simulink model "arducopter"  (R2024b)
settings: Solver=FixedStepAuto  StartTime=0.0  StopTime=simIn.param.timeEnd  FixedStep=simIn.param.dt  RelTol=1e-3
undefined symbols (not defined in the file or in its folder): DiscIntNeverNeededParam, sim, simIn
libraries: simulink x60, slident x4, vrlib x1
(part 5 of 9)

== system arducopter/Position Controller/PID Velocity z/I ==
  note: Integrator, see AC_PID_Basic::update_i()
      | Initialization: integrator=0 (see AC_PosControl::init_z())
  e : Inport
  limitNeg : Inport  Port=2
  limitPos : Inport  Port=3
  ki : Inport  Port=4
  i_max : Inport  Port=5
  Constant1 : Constant  Value=simIn.param.dt
  Data Type Conversion1 : DataTypeConversion  OutDataTypeStr=single  SaturateOnIntegerOverflow=off  RndMeth=Floor
  IC1 : InitialCondition  Value=0
  Integrator : MATLAB Function  TreatAsAtomicUnit=on
  Unit Delay1 : UnitDelay  InitialCondition=single(0)  SampleTime=-1  HasFrameUpgradeWarning=on
  integrator : Outport
  wires:
  e/1 -> Integrator/1(error)
  Integrator/1(integrator_out) -> IC1/1
  [integrator_out] -> integrator/1
  Constant1/1 -> Data Type Conversion1/1
  limitNeg/1 -> Integrator/3(limitNeg)
  [integrator_out] -> Unit Delay1/1
  IC1/1 -> [integrator_out]
  Unit Delay1/1 -> Integrator/2(integrator)
  ki/1 -> Integrator/5(ki)
  i_max/1 -> Integrator/6(i_max)
  Data Type Conversion1/1 -> Integrator/7(dt)
  limitPos/1 -> Integrator/4(limitPos)

== system arducopter/Position Controller/PID Velocity z/RAT_FLTD ==
  note: Digital Filter:
      | $y_n = (1 - \alpha)y_{n-1} + x \cdot \alpha$
  note: Alpha Calculation:
      | $\alpha = \frac{\mathrm{d}t}{\mathrm{d}t + 2 \pi f_{\mathrm{Cutoff}}$
  note: See AC_PID_Basics.cpp, update_all()
  note: See AP_Math.cpp, calc_lowpass_alpha_dt()
  u : Inport
  cutoff_freq : Inport  Port=2
  ATC input time constant : Constant  Value=simIn.param.dt
  Add : Sum
  Calculate Alpha : Product  Inputs=*/
  Compare To Zero : simulink/Logic and Bit Operations/Compare To Zero  relop=<=  OutDataTypeStr=boolean
  Compare To Zero1 : simulink/Logic and Bit Operations/Compare To Zero  relop=<=  OutDataTypeStr=boolean
  Constant2 : Constant  OutDataTypeStr=single
  Constant3 : Constant  OutDataTypeStr=single
  Constant4 : Constant  OutDataTypeStr=single
  Data Type Conversion1 : DataTypeConversion  OutDataTypeStr=single  SaturateOnIntegerOverflow=off  RndMeth=Floor
  Divide : Product  Inputs=*/
  Gain : Gain  Gain=2*pi
  IC : InitialCondition  Value=0
  Logical Operator : Logic  Operator=OR  AllPortsSameDT=off  OutDataTypeStr=boolean
  Product : Product
  Product1 : Product
  Subtract1 : Sum  Inputs=+-
  Sum : Sum  Inputs=++|  OutDataTypeStr=single
  Switch : Switch  Criteria=u2 > Threshold  SaturateOnIntegerOverflow=off  InputSameDT=off
  Unit Delay : UnitDelay  SampleTime=-1  HasFrameUpgradeWarning=on
  y : Outport
  wires:
  Product1/1 -> Sum/2
  Unit Delay/1 -> Product1/2
  Subtract1/1 -> Product1/1
  [alpha] -> Subtract1/2
  Constant2/1 -> Subtract1/1
  [alpha] -> Product/1
  Calculate Alpha/1 -> Switch/3
  Add/1 -> Calculate Alpha/2
  [dt] -> Add/1, Calculate Alpha/1
  Gain/1 -> Divide/2
  cutoff_freq/1 -> [cutoff_freq]
  u/1 -> Product/2
  Divide/1 -> Add/2
  Constant3/1 -> Divide/1
  Product/1 -> Sum/1
  Switch/1 -> [alpha]
  ATC input time constant/1 -> Data Type Conversion1/1
  [cutoff_freq] -> Gain/1
  [dt] -> Compare To Zero/1
  [cutoff_freq] -> Compare To Zero1/1
  Compare To Zero/1 -> Logical Operator/1
  Compare To Zero1/1 -> Logical Operator/2
  Logical Operator/1 -> Switch/2
  Constant4/1 -> Switch/1
  Sum/1 -> IC/1
  IC/1 -> Unit Delay/1, y/1
  Data Type Conversion1/1 -> [dt]

== system arducopter/Position Controller/PID Velocity z/RAT_FLTE ==
  note: Digital Filter:
      | $y_n = (1 - \alpha)y_{n-1} + x \cdot \alpha$
  note: Alpha Calculation:
      | $\alpha = \frac{\mathrm{d}t}{\mathrm{d}t + 2 \pi f_{\mathrm{Cutoff}}$
  note: See AC_PID_Basic.cpp, update_all()
  note: See AP_Math.cpp, calc_lowpass_alpha_dt()
  u : Inport
  cutoff_freq : Inport  Port=2
  ATC input time constant : Constant  Value=simIn.param.dt
  Add : Sum
  Calculate Alpha : Product  Inputs=*/
  Compare To Zero : simulink/Logic and Bit Operations/Compare To Zero  relop=<=  OutDataTypeStr=boolean
  Compare To Zero1 : simulink/Logic and Bit Operations/Compare To Zero  relop=<=  OutDataTypeStr=boolean
  Constant2 : Constant  OutDataTypeStr=single
  Constant3 : Constant  OutDataTypeStr=single
  Constant4 : Constant  OutDataTypeStr=single
  Data Type Conversion1 : DataTypeConversion  OutDataTypeStr=single  SaturateOnIntegerOverflow=off  RndMeth=Floor
  Divide : Product  Inputs=*/
  Gain : Gain  Gain=2*pi
  IC : InitialCondition  Value=0
  Logical Operator : Logic  Operator=OR  AllPortsSameDT=off  OutDataTypeStr=boolean
  Product : Product
  Product1 : Product
  Subtract1 : Sum  Inputs=+-
  Sum : Sum  Inputs=++|  OutDataTypeStr=single
  Switch : Switch  Criteria=u2 > Threshold  SaturateOnIntegerOverflow=off  InputSameDT=off
  Unit Delay : UnitDelay  SampleTime=-1  HasFrameUpgradeWarning=on
  y : Outport
  wires:
  Product1/1 -> Sum/2
  Unit Delay/1 -> Product1/2
  Subtract1/1 -> Product1/1
  [alpha] -> Subtract1/2
  Constant2/1 -> Subtract1/1
  [alpha] -> Product/1
  Calculate Alpha/1 -> Switch/3
  Add/1 -> Calculate Alpha/2
  [dt] -> Add/1, Calculate Alpha/1
  Gain/1 -> Divide/2
  cutoff_freq/1 -> [cutoff_freq]
  u/1 -> Product/2
  Divide/1 -> Add/2
  Constant3/1 -> Divide/1
  Product/1 -> Sum/1
  Switch/1 -> [alpha]
  ATC input time constant/1 -> Data Type Conversion1/1
  [cutoff_freq] -> Gain/1
  [dt] -> Compare To Zero/1
  [cutoff_freq] -> Compare To Zero1/1
  Compare To Zero/1 -> Logical Operator/1
  Compare To Zero1/1 -> Logical Operator/2
  Logical Operator/1 -> Switch/2
  Constant4/1 -> Switch/1
  Sum/1 -> IC/1
  IC/1 -> Unit Delay/1, y/1
  Data Type Conversion1/1 -> [dt]

== system arducopter/Position Controller/PID Velocity z/Scale Factor Z ==
  note: AP_AHRS::getControlScaleZ()
      | This subsystem calculates a scaling factor for the target of vertical motion quantities based on the EKF type that is being used.
      | Taken from AP_AHRS::getControlScaleZ() in AP_AHRS.cpp. Called in AC_PosControl::update_z_controller().
      | Flying with only DCM lower the gain of the controllers by 4x to cope with high lag.
  ekfType : Inport
  EKF used : Constant  OutDataTypeStr=single
  No EKF : Constant  Value=0.25  OutDataTypeStr=single
  Switch : Switch  Criteria=u2 > Threshold  SaturateOnIntegerOverflow=off  InputSameDT=off
  scale_z : Outport
  wires:
  ekfType/1 -> Switch/2
  EKF used/1 -> Switch/1
  No EKF/1 -> Switch/3
  Switch/1 -> scale_z/1

== system arducopter/Position Controller/calc des climb rate/constrain climb rate ==
  note: Based on get_pilot_speed_dn()
      | Use maximum up-speed if down-speed limit is 0
  in : Inport
  Abs : Abs  SaturateOnIntegerOverflow=off
  Abs1 : Abs  SaturateOnIntegerOverflow=off
  Constant1 : Constant  Value=simIn.param.PSCD.VEL_MAX_DN
  Constant2 : Constant  Value=simIn.param.PSCD.VEL_MAX_UP
  Constant3 : Constant  Value=simIn.param.PSCD.VEL_MAX_UP
  Gain : Gain  Gain=-1
  Saturation Dynamic : simulink/Discontinuities/Saturation Dynamic  OutMin=[]  OutMax=[]  OutDataTypeStr=Inherit: Same as second input  OutDataType=fixdt(1, 16)  OutScaling=2^-10  DoSatur=off
  Switch : Switch  Criteria=u2 > Threshold  SaturateOnIntegerOverflow=off  InputSameDT=off
  out : Outport
  wires:
  Constant1/1 -> Abs/1, Switch/2
  Constant2/1 -> Abs1/1
  Abs/1 -> Switch/1
  Abs1/1 -> Switch/3
  Saturation Dynamic/1 -> out/1
  Switch/1 -> Gain/1
  Gain/1 -> Saturation Dynamic/3
  in/1 -> Saturation Dynamic/2
  Constant3/1 -> Saturation Dynamic/1

== system arducopter/Position Controller/set_pos_target_z_from_climb_rate()/input_vel_accel_z ==
  note: input_vel_accel_z()
      | This subsystem takes the current target position (posTarIn) and desired velocity and acceleration (velDesTar and accDesTar).
      | First, it updates the target position and desired velocity based on the current desired acceleration (accDesIn) (1).
      | Secondly, it calculates the required jerk limited adjustment to the acceleration for the next time dt (accDes) to reach the desired velocity and acceleration targets (velDesTar and accDesTar) (2).
  note: (2) shape_vel_accel()
      | Adjustment of the desired acceleration to follow a jerk limited kinematic path to vel and acc
  note: (1) update_pos_vel_accel()
      | Adjust desired position and velocity based on desired acceleration
  note: Calculate overspeed gain to calculate increased max accel and jerk if over speed
  velDesTar : Inport
  accDesTar : Inport  Port=2
  limitVectorZ : Inport  Port=3
  velMaxUp : Inport  Port=4
  velMaxDn : Inport  Port=5
  accMaxZ : Inport  Port=6
  jerkMax : Inport  Port=7
  posTarIn : Inport  Port=8
  posErr : Inport  Port=9
  velErr : Inport  Port=10
  velDesIn : Inport  Port=11
  accDesIn : Inport  Port=12
  Constant : Constant  Value=simIn.param.PSCD.OVERSPEED_GAIN_Z
  Constant1 : Constant  OutDataTypeStr=boolean
  Constant2 : Constant  Value=simIn.param.dt  OutDataTypeStr=single
  MATLAB Function : MATLAB Function  TreatAsAtomicUnit=on
  Product : Product
  Product1 : Product
  calc accMin : Subsystem
  shape_vel_accel : Subsystem
  update_pos_vel_accel : Subsystem
  posTar : Outport
  velDes : Outport  Port=2
  accDes : Outport  Port=3
  wires:
  velMaxUp/1 -> MATLAB Function/1(velMaxUp)
  accMaxZ/1 -> Product/2
  velDesIn/1 -> [velDesIn]
  velMaxDn/1 -> MATLAB Function/2(velMaxDn)
  Constant/1 -> MATLAB Function/4(overspeedGainDefault)
  [velDesIn] -> MATLAB Function/3(velDes)
  posTarIn/1 -> update_pos_vel_accel/1(posTarIn)
  [velDesIn] -> update_pos_vel_accel/2(velDesIn)
  accDesIn/1 -> [accDesIn]
  limitVectorZ/1 -> update_pos_vel_accel/4(limitVectorZ)
  update_pos_vel_accel/2(velDes) -> [velDes]
  accDesTar/1 -> shape_vel_accel/2(acc)
  velDesTar/1 -> shape_vel_accel/1(vel)
  [accDesIn] -> update_pos_vel_accel/3(accDesIn)
  [accDesIn] -> shape_vel_accel/4(accDes)
  [accMax] -> calc accMin/1(accMax), shape_vel_accel/6(accMax)
  calc accMin/1(accMin) -> shape_vel_accel/5(accMin)
  Constant2/1 -> shape_vel_accel/8(dt)
  Constant1/1 -> shape_vel_accel/9(limitTotalAccel)
  update_pos_vel_accel/1(posTar) -> posTar/1
  [velDes] -> shape_vel_accel/3(velDes)
  [velDes] -> velDes/1
  shape_vel_accel/1(accDesShaped) -> accDes/1
  MATLAB Function/1(overspeedGain) -> Product1/1, Product/1
  Product/1 -> [accMax]
  jerkMax/1 -> Product1/2
  Product1/1 -> [jerkMax]
  [jerkMax] -> shape_vel_accel/7(jerkMax)
  posErr/1 -> update_pos_vel_accel/5(posErr)
  velErr/1 -> update_pos_vel_accel/6(velErr)

== system arducopter/Rate Controller/PID Pitch Rate/Calc Derivative ==
  e : Inport
  ATC input time constant : Constant  Value=simIn.param.dt
  Data Type Conversion : DataTypeConversion  OutDataTypeStr=single  SaturateOnIntegerOverflow=off  RndMeth=Floor
  Divide : Product  Inputs=*/
  Sum : Sum  Inputs=|+-
  Unit Delay : UnitDelay  SampleTime=-1  HasFrameUpgradeWarning=on
  derivative : Outport
  wires:
  e/1 -> Sum/1, Unit Delay/1
  Unit Delay/1 -> Sum/2
  Sum/1 -> Divide/1
  ATC input time constant/1 -> Data Type Conversion/1
  Divide/1 -> derivative/1
  Data Type Conversion/1 -> Divide/2

== system arducopter/Rate Controller/PID Pitch Rate/I ==
  note: Integrator, see AC_PID::update_i()
  e : Inport
  limit_flg : Inport  Port=2
  ki : Inport  Port=3
  i_max : Inport  Port=4
  Constant1 : Constant  Value=simIn.param.dt
  Data Type Conversion : DataTypeConversion  OutDataTypeStr=single  SaturateOnIntegerOverflow=off  RndMeth=Floor
  IC1 : InitialCondition  Value=simIn.init.PIDP.I
  Integrator : MATLAB Function  TreatAsAtomicUnit=on
  Unit Delay1 : UnitDelay  SampleTime=-1  HasFrameUpgradeWarning=on
  integrator : Outport
  wires:
  [integrator_out] -> integrator/1
  Constant1/1 -> Data Type Conversion/1
  limit_flg/1 -> Integrator/3(limit_flg)
  [integrator_out] -> Unit Delay1/1
  IC1/1 -> [integrator_out]
  Unit Delay1/1 -> Integrator/2(integrator)
  ki/1 -> Integrator/4(ki)
  i_max/1 -> Integrator/5(i_max)
  e/1 -> Integrator/1(error)
  Integrator/1(integrator_out) -> IC1/1
  Data Type Conversion/1 -> Integrator/6(dt)

== system arducopter/Rate Controller/PID Pitch Rate/RAT_FLTD ==
  note: Digital Filter:
      | $y_n = (1 - \alpha)y_{n-1} + x \cdot \alpha$
  note: See AC_PID.cpp, update_all()
  note: See AP_Math.cpp, calc_lowpass_alpha_dt()
  note: Alpha Calculation:
      | $\alpha = \frac{\mathrm{d}t}{\mathrm{d}t + 2 \pi f_{\mathrm{Cutoff}}$
  u : Inport
  cutoff_freq : Inport  Port=2
  ATC input time constant1 : Constant  Value=simIn.param.dt
  Add1 : Sum
  Calculate Alpha1 : Product  Inputs=*/
  Compare To Zero2 : simulink/Logic and Bit Operations/Compare To Zero  relop=<=  OutDataTypeStr=boolean
  Compare To Zero3 : simulink/Logic and Bit Operations/Compare To Zero  relop=<=  OutDataTypeStr=boolean
  Compare To Zero4 : simulink/Logic and Bit Operations/Compare To Zero  relop=~=  OutDataTypeStr=boolean
  Constant1 : Constant  OutDataTypeStr=single
  Constant2 : Constant  OutDataTypeStr=single
  Constant5 : Constant  OutDataTypeStr=single
  Data Type Conversion1 : DataTypeConversion  OutDataTypeStr=single  SaturateOnIntegerOverflow=off  RndMeth=Floor
  Divide1 : Product  Inputs=*/
  Gain1 : Gain  Gain=2*pi
  IC : InitialCondition  Value=simIn.init.PIDP.DerFilt
  Logical Operator1 : Logic  Operator=OR  AllPortsSameDT=off  OutDataTypeStr=boolean
  Product : Product
  Product1 : Product
  Product2 : Product
  Subtract1 : Sum  Inputs=+-
  Sum : Sum  Inputs=++|  AccumDataTypeStr=single
  Switch1 : Switch  Criteria=u2 > Threshold  SaturateOnIntegerOverflow=off  InputSameDT=off
  Unit Delay : UnitDelay  SampleTime=-1  HasFrameUpgradeWarning=on
  y : Outport
  wires:
  Product1/1 -> Sum/2
  Unit Delay/1 -> Product1/2
  Subtract1/1 -> Product1/1
  [alpha] -> Subtract1/2
  Constant2/1 -> Subtract1/1
  [alpha] -> Product/1
  u/1 -> Product/2
  Product/1 -> Sum/1
  Sum/1 -> IC/1
  IC/1 -> Unit Delay/1, y/1
  [dt] -> Compare To Zero2/1
  Constant1/1 -> Divide1/1
  Divide1/1 -> Add1/2
  Product2/1 -> Switch1/1
  Add1/1 -> Calculate Alpha1/2
  Gain1/1 -> Divide1/2
  Compare To Zero3/1 -> Logical Operator1/2
  [dt] -> Compare To Zero4/1
  Data Type Conversion1/1 -> [dt]
  ATC input time constant1/1 -> Data Type Conversion1/1
  [cutoff_freq] -> Gain1/1
  Switch1/1 -> [alpha]
  [dt] -> Calculate Alpha1/1, Add1/1
  Compare To Zero4/1 -> Product2/1
  cutoff_freq/1 -> [cutoff_freq]
  Compare To Zero2/1 -> Logical Operator1/1
  [cutoff_freq] -> Compare To Zero3/1
  Calculate Alpha1/1 -> Switch1/3
  Logical Operator1/1 -> Switch1/2
  Constant5/1 -> Product2/2

== system arducopter/Rate Controller/PID Pitch Rate/RAT_FLTE ==
  note: Digital Filter:
      | $y_n = (1 - \alpha)y_{n-1} + x \cdot \alpha$
  note: See AC_PID.cpp, update_all()
  note: See AP_Math.cpp, calc_lowpass_alpha_dt()
  note: Alpha Calculation:
      | $\alpha = \frac{\mathrm{d}t}{\mathrm{d}t + 2 \pi f_{\mathrm{Cutoff}}$
  u : Inport
  cutoff_freq : Inport  Port=2
  ATC input time constant1 : Constant  Value=simIn.param.dt
  Add1 : Sum
  Calculate Alpha1 : Product  Inputs=*/
  Compare To Zero2 : simulink/Logic and Bit Operations/Compare To Zero  relop=<=  OutDataTypeStr=boolean
  Compare To Zero3 : simulink/Logic and Bit Operations/Compare To Zero  relop=<=  OutDataTypeStr=boolean
  Compare To Zero4 : simulink/Logic and Bit Operations/Compare To Zero  relop=~=  OutDataTypeStr=boolean
  Constant1 : Constant  OutDataTypeStr=single
  Constant2 : Constant  OutDataTypeStr=single
  Constant5 : Constant  OutDataTypeStr=single
  Data Type Conversion1 : DataTypeConversion  OutDataTypeStr=single  SaturateOnIntegerOverflow=off  RndMeth=Floor
  Divide1 : Product  Inputs=*/
  Gain1 : Gain  Gain=2*pi
  IC : InitialCondition  Value=simIn.init.PIDP.ErrFilt
  Logical Operator1 : Logic  Operator=OR  AllPortsSameDT=off  OutDataTypeStr=boolean
  Product : Product
  Product1 : Product
  Product2 : Product
  Subtract1 : Sum  Inputs=+-
  Sum : Sum  Inputs=++|  OutDataTypeStr=single
  Switch1 : Switch  Criteria=u2 > Threshold  SaturateOnIntegerOverflow=off  InputSameDT=off
  Unit Delay : UnitDelay  SampleTime=-1  HasFrameUpgradeWarning=on
  y : Outport
  wires:
  Product1/1 -> Sum/2
  Unit Delay/1 -> Product1/2
  Subtract1/1 -> Product1/1
  [alpha] -> Subtract1/2
  Constant2/1 -> Subtract1/1
  [alpha] -> Product/1
  u/1 -> Product/2
  Product/1 -> Sum/1
  Sum/1 -> IC/1
  IC/1 -> Unit Delay/1, y/1
  [dt] -> Compare To Zero2/1
  Constant1/1 -> Divide1/1
  Divide1/1 -> Add1/2
  Product2/1 -> Switch1/1
  Add1/1 -> Calculate Alpha1/2
  Gain1/1 -> Divide1/2
  Compare To Zero3/1 -> Logical Operator1/2
  [dt] -> Compare To Zero4/1
  Data Type Conversion1/1 -> [dt]
  ATC input time constant1/1 -> Data Type Conversion1/1
  [cutoff_freq] -> Gain1/1
  Switch1/1 -> [alpha]
  [dt] -> Calculate Alpha1/1, Add1/1
  Compare To Zero4/1 -> Product2/1
  cutoff_freq/1 -> [cutoff_freq]
  Compare To Zero2/1 -> Logical Operator1/1
  [cutoff_freq] -> Compare To Zero3/1
  Calculate Alpha1/1 -> Switch1/3
  Logical Operator1/1 -> Switch1/2
  Constant5/1 -> Product2/2

== system arducopter/Rate Controller/PID Pitch Rate/RAT_FLTT ==
  note: See AC_PID.cpp, update_all()
  note: Digital Filter:
      | $y_n = (1 - \alpha)y_{n-1} + x \cdot \alpha$
  note: Alpha Calculation:
      | $\alpha = \frac{\mathrm{d}t}{\mathrm{d}t + 2 \pi f_{\mathrm{Cutoff}}$
  note: See AP_Math.cpp, calc_lowpass_alpha_dt()
  u : Inport
  cutoff_freq : Inport  Port=2
  ATC input time constant1 : Constant  Value=simIn.param.dt
  Add1 : Sum
  Calculate Alpha1 : Product  Inputs=*/
  Compare To Zero2 : simulink/Logic and Bit Operations/Compare To Zero  relop=<=  OutDataTypeStr=boolean
  Compare To Zero3 : simulink/Logic and Bit Operations/Compare To Zero  relop=<=  OutDataTypeStr=boolean
  Compare To Zero4 : simulink/Logic and Bit Operations/Compare To Zero  relop=~=  OutDataTypeStr=boolean
  Constant1 : Constant  OutDataTypeStr=single
  Constant2 : Constant  OutDataTypeStr=single
  Constant5 : Constant  OutDataTypeStr=single
  Data Type Conversion1 : DataTypeConversion  OutDataTypeStr=single  SaturateOnIntegerOverflow=off  RndMeth=Floor
  Divide1 : Product  Inputs=*/
  Gain1 : Gain  Gain=2*pi
  IC : InitialCondition  Value=simIn.init.PIDP.TarFilt
  Logical Operator1 : Logic  Operator=OR  AllPortsSameDT=off  OutDataTypeStr=boolean
  Product : Product
  Product1 : Product
  Product2 : Product
  Subtract1 : Sum  Inputs=+-
  Sum : Sum  Inputs=++|
  Switch1 : Switch  Criteria=u2 > Threshold  SaturateOnIntegerOverflow=off  InputSameDT=off
  Unit Delay : UnitDelay  SampleTime=-1  HasFrameUpgradeWarning=on
  y : Outport
  wires:
  Product/1 -> Sum/1
  u/1 -> Product/2
  [alpha] -> Product/1
  Constant2/1 -> Subtract1/1
  [alpha] -> Subtract1/2
  Subtract1/1 -> Product1/1
  Product1/1 -> Sum/2
  Sum/1 -> IC/1
  Unit Delay/1 -> Product1/2
  IC/1 -> y/1, Unit Delay/1
  Add1/1 -> Calculate Alpha1/2
  Constant1/1 -> Divide1/1
  Compare To Zero2/1 -> Logical Operator1/1
  Logical Operator1/1 -> Switch1/2
  cutoff_freq/1 -> [cutoff_freq]
  Switch1/1 -> [alpha]
  [dt] -> Calculate Alpha1/1, Add1/1
  [cutoff_freq] -> Compare To Zero3/1
  Compare To Zero3/1 -> Logical Operator1/2
  Data Type Conversion1/1 -> [dt]
  [cutoff_freq] -> Gain1/1
  [dt] -> Compare To Zero2/1
  Divide1/1 -> Add1/2
  Gain1/1 -> Divide1/2
  ATC input time constant1/1 -> Data Type Conversion1/1
  Calculate Alpha1/1 -> Switch1/3
  [dt] -> Compare To Zero4/1
  Product2/1 -> Switch1/1
  Constant5/1 -> Product2/2
  Compare To Zero4/1 -> Product2/1

== system arducopter/Rate Controller/PID Pitch Rate/Slew Limiter ==
  note: Data Store Memory Elements: Global variables of subsystem
  note: Slew Limiter
      |
      | Calculates the slew limit modifiert Dmod for the P and D part of the controller. The calculation of Dmod is taken from SlewLimiter::modifier() in SlewLimiter.cpp.
  note: Alpha Calculation:
      | $\alpha = \frac{\mathrm{d}t}{\mathrm{d}t + 2 \pi f_{\mathrm{Cutoff}}$
  note: See AP_Math.cpp, calc_lowpass_alpha_dt()
  p_out : Inport
  sr_max : Inport  Port=2
  sr_tau : Inport  Port=3
  sr_flt_f : Inport  Port=4
  clock : Inport  Port=5
  d_out : Inport  Port=6
  ATC input time constant : Constant  Value=simIn.param.dt
  Add1 : Sum
  Calculate Alpha : Product  Inputs=*/
  Calculate Dmod : MATLAB Function  TreatAsAtomicUnit=on  SystemSampleTime=0.0025
  Compare To Zero2 : simulink/Logic and Bit Operations/Compare To Zero  relop=<=  OutDataTypeStr=boolean
  Compare To Zero3 : simulink/Logic and Bit Operations/Compare To Zero  relop=<=  OutDataTypeStr=boolean
  Compare To Zero4 : simulink/Logic and Bit Operations/Compare To Zero  relop=~=  OutDataTypeStr=boolean
  Constant1 : Constant  OutDataTypeStr=single
  Constant5 : Constant  OutDataTypeStr=single
  Data Store Memory : DataStoreMemory  DataStoreName=pos_event_stored  ReadBeforeWriteMsg=warning  WriteAfterWriteMsg=warning  WriteAfterReadMsg=warning  InitialValue=false  ShowAdditionalParam=off  OutDataTypeStr=boolean
  Data Store Memory1 : DataStoreMemory  DataStoreName=neg_event_stored  ReadBeforeWriteMsg=warning  WriteAfterWriteMsg=warning  WriteAfterReadMsg=warning  InitialValue=false  ShowAdditionalParam=off  OutDataTypeStr=boolean
  Data Store Memory10 : DataStoreMemory  DataStoreName=modifier_slew_rate  ReadBeforeWriteMsg=warning  WriteAfterWriteMsg=warning  WriteAfterReadMsg=warning  InitialValue=simIn.init.PIDP.SROut  ShowAdditionalParam=off  OutDataTypeStr=single
  Data Store Memory11 : DataStoreMemory  DataStoreName=output_slew_rate  ReadBeforeWriteMsg=warning  WriteAfterWriteMsg=warning  WriteAfterReadMsg=warning  InitialValue=simIn.init.PIDP.SROut  ShowAdditionalParam=off  OutDataTypeStr=single
  Data Store Memory2 : DataStoreMemory  DataStoreName=pos_event_idx  ReadBeforeWriteMsg=warning  WriteAfterWriteMsg=warning  WriteAfterReadMsg=warning  InitialValue=1  ShowAdditionalParam=off  OutDataTypeStr=int8
  Data Store Memory3 : DataStoreMemory  DataStoreName=neg_event_idx  ReadBeforeWriteMsg=warning  WriteAfterWriteMsg=warning  WriteAfterReadMsg=warning  InitialValue=1  ShowAdditionalParam=off  OutDataTypeStr=int8
  Data Store Memory4 : DataStoreMemory  DataStoreName=pos_event_ms  ReadBeforeWriteMsg=warning  WriteAfterWriteMsg=warning  WriteAfterReadMsg=warning  InitialValue=[0 0]  ShowAdditionalParam=off  OutDataTypeStr=uint32  Dimensions=2
  Data Store Memory5 : DataStoreMemory  DataStoreName=neg_event_ms  ReadBeforeWriteMsg=warning  WriteAfterWriteMsg=warning  WriteAfterReadMsg=warning  InitialValue=[0 0]  ShowAdditionalParam=off  OutDataTypeStr=uint32  Dimensions=2
  Data Store Memory6 : DataStoreMemory  DataStoreName=max_pos_slew_rate  ReadBeforeWriteMsg=warning  WriteAfterWriteMsg=warning  WriteAfterReadMsg=warning  ShowAdditionalParam=off  OutDataTypeStr=single
  Data Store Memory7 : DataStoreMemory  DataStoreName=max_pos_slew_event_ms  ReadBeforeWriteMsg=warning  WriteAfterWriteMsg=warning  WriteAfterReadMsg=warning  ShowAdditionalParam=off  OutDataTypeStr=uint32
  Data Store Memory8 : DataStoreMemory  DataStoreName=max_neg_slew_rate  ReadBeforeWriteMsg=warning  WriteAfterWriteMsg=warning  WriteAfterReadMsg=warning  ShowAdditionalParam=off  OutDataTypeStr=single
  Data Store Memory9 : DataStoreMemory  DataStoreName=max_neg_slew_event_ms  ReadBeforeWriteMsg=warning  WriteAfterWriteMsg=warning  WriteAfterReadMsg=warning  ShowAdditionalParam=off  OutDataTypeStr=uint32
  Data Store Read : DataStoreRead  DataStoreName=modifier_slew_rate  DataStoreElements=modifier_slew_rate  IndexOptions=Index vector (dialog)  Indices=1  OutputSizes=1
  Data Store Read1 : DataStoreRead  DataStoreName=output_slew_rate  DataStoreElements=output_slew_rate  IndexOptions=Index vector (dialog)  Indices=1  OutputSizes=1
  Data Type Conversion2 : DataTypeConversion  OutDataTypeStr=single  SaturateOnIntegerOverflow=off  RndMeth=Floor
  Divide1 : Product  Inputs=*/
  Gain1 : Gain  Gain=2*pi
  IC : InitialCondition  Value=2*simIn.init.PIDP.SROut
  Logical Operator1 : Logic  Operator=OR  AllPortsSameDT=off  OutDataTypeStr=boolean
  Lowpass Filter : MATLAB Function  TreatAsAtomicUnit=on
  Product2 : Product
  Subsystem : Subsystem
  Switch1 : Switch  Criteria=u2 > Threshold  SaturateOnIntegerOverflow=off  InputSameDT=off
  Terminator : Terminator
  Terminator1 : Terminator
  Unit Delay1 : UnitDelay  SampleTime=-1  HasFrameUpgradeWarning=on
  Dmod : Outport
  wires:
  Lowpass Filter/1(out) -> IC/1  "pitchRateSrFilt"
  Unit Delay1/1 -> Lowpass Filter/3(out_last)
  Calculate Dmod/1(Dmod) -> Dmod/1  "pitchRateDmod"
  sr_max/1 -> Calculate Dmod/2(sr_max)
  sr_tau/1 -> Calculate Dmod/3(sr_tau)
  Data Store Read/1 -> Terminator/1  "pitchRateSrModifier"
  Data Store Read1/1 -> Terminator1/1  "pitchRateSrOut"
  p_out/1 -> Subsystem/1(p_out)
  d_out/1 -> Subsystem/2(d_out)
  Subsystem/1(sr_raw) -> Lowpass Filter/1(in)  "pitchRateSrRaw"
  IC/1 -> Calculate Dmod/1(slew_rate), Unit Delay1/1
  clock/1 -> Calculate Dmod/5(time)
  [cutoff_freq] -> Gain1/1
  [dt] -> Calculate Alpha/1, Add1/1
  Calculate Alpha/1 -> Switch1/3
  Gain1/1 -> Divide1/2
  Data Type Conversion2/1 -> [dt]
  ATC input time constant/1 -> Data Type Conversion2/1
  [cutoff_freq] -> Compare To Zero3/1
  Compare To Zero3/1 -> Logical Operator1/2
  Constant1/1 -> Divide1/1
  [dt] -> Compare To Zero2/1
  Logical Operator1/1 -> Switch1/2
  Compare To Zero2/1 -> Logical Operator1/1
  Add1/1 -> Calculate Alpha/2
  Divide1/1 -> Add1/2
  Product2/1 -> Switch1/1
  [dt] -> Compare To Zero4/1
  Switch1/1 -> Lowpass Filter/2(alpha)
  Compare To Zero4/1 -> Product2/1
  Constant5/1 -> Product2/2
  sr_flt_f/1 -> [cutoff_freq]
  [dt] -> Calculate Dmod/4(dt)

== system arducopter/Rate Controller/PID Roll Rate/Calc Derivative ==
  e : Inport
  ATC input time constant : Constant  Value=simIn.param.dt
  Data Type Conversion : DataTypeConversion  OutDataTypeStr=single  SaturateOnIntegerOverflow=off  RndMeth=Floor
  Divide : Product  Inputs=*/
  Sum : Sum  Inputs=|+-
  Unit Delay : UnitDelay  SampleTime=-1  HasFrameUpgradeWarning=on
  derivative : Outport
  wires:
  e/1 -> Sum/1, Unit Delay/1
  Unit Delay/1 -> Sum/2
  Sum/1 -> Divide/1
  ATC input time constant/1 -> Data Type Conversion/1
  Divide/1 -> derivative/1
  Data Type Conversion/1 -> Divide/2

== system arducopter/Rate Controller/PID Roll Rate/I ==
  note: Integrator, see AC_PID::update_i()
  e : Inport
  limit_flg : Inport  Port=2
  ki : Inport  Port=3
  i_max : Inport  Port=4
  Constant1 : Constant  Value=simIn.param.dt
  Data Type Conversion : DataTypeConversion  OutDataTypeStr=single  SaturateOnIntegerOverflow=off  RndMeth=Floor
  IC1 : InitialCondition  Value=simIn.init.PIDR.I
  Integrator : MATLAB Function  TreatAsAtomicUnit=on
  Unit Delay1 : UnitDelay  SampleTime=-1  HasFrameUpgradeWarning=on
  integrator : Outport
  wires:
  [integrator_out] -> integrator/1
  Constant1/1 -> Data Type Conversion/1
  limit_flg/1 -> Integrator/3(limit_flg)
  [integrator_out] -> Unit Delay1/1
  IC1/1 -> [integrator_out]
  Unit Delay1/1 -> Integrator/2(integrator)
  ki/1 -> Integrator/4(ki)
  i_max/1 -> Integrator/5(i_max)
  e/1 -> Integrator/1(error)
  Integrator/1(integrator_out) -> IC1/1
  Data Type Conversion/1 -> Integrator/6(dt)

== system arducopter/Rate Controller/PID Roll Rate/RAT_FLTD ==
  note: Digital Filter:
      | $y_n = (1 - \alpha)y_{n-1} + x \cdot \alpha$
  note: See AC_PID.cpp, update_all()
  note: See AP_Math.cpp, calc_lowpass_alpha_dt()
  note: Alpha Calculation:
      | $\alpha = \frac{\mathrm{d}t}{\mathrm{d}t + 2 \pi f_{\mathrm{Cutoff}}$
  u : Inport
  cutoff_freq : Inport  Port=2
  ATC input time constant1 : Constant  Value=simIn.param.dt
  Add1 : Sum
  Calculate Alpha1 : Product  Inputs=*/
  Compare To Zero2 : simulink/Logic and Bit Operations/Compare To Zero  relop=<=  OutDataTypeStr=boolean
  Compare To Zero3 : simulink/Logic and Bit Operations/Compare To Zero  relop=<=  OutDataTypeStr=boolean
  Compare To Zero4 : simulink/Logic and Bit Operations/Compare To Zero  relop=~=  OutDataTypeStr=boolean
  Constant1 : Constant  OutDataTypeStr=single
  Constant2 : Constant  OutDataTypeStr=single
  Constant5 : Constant  OutDataTypeStr=single
  Data Type Conversion1 : DataTypeConversion  OutDataTypeStr=single  SaturateOnIntegerOverflow=off  RndMeth=Floor
  Divide1 : Product  Inputs=*/
  Gain1 : Gain  Gain=2*pi
  IC : InitialCondition  Value=simIn.init.PIDR.DerFilt
  Logical Operator1 : Logic  Operator=OR  AllPortsSameDT=off  OutDataTypeStr=boolean
  Product : Product
  Product1 : Product
  Product2 : Product
  Subtract1 : Sum  Inputs=+-
  Sum : Sum  Inputs=++|  AccumDataTypeStr=single
  Switch1 : Switch  Criteria=u2 > Threshold  SaturateOnIntegerOverflow=off  InputSameDT=off
  Unit Delay : UnitDelay  SampleTime=-1  HasFrameUpgradeWarning=on
  y : Outport
  wires:
  Product1/1 -> Sum/2
  Unit Delay/1 -> Product1/2
  Subtract1/1 -> Product1/1
  [alpha] -> Subtract1/2
  Constant2/1 -> Subtract1/1
  [alpha] -> Product/1
  u/1 -> Product/2
  Product/1 -> Sum/1
  Sum/1 -> IC/1
  IC/1 -> Unit Delay/1, y/1
  [dt] -> Compare To Zero2/1
  Constant1/1 -> Divide1/1
  Divide1/1 -> Add1/2
  Product2/1 -> Switch1/1
  Add1/1 -> Calculate Alpha1/2
  Gain1/1 -> Divide1/2
  Compare To Zero3/1 -> Logical Operator1/2
  [dt] -> Compare To Zero4/1
  Data Type Conversion1/1 -> [dt]
  ATC input time constant1/1 -> Data Type Conversion1/1
  [cutoff_freq] -> Gain1/1
  Switch1/1 -> [alpha]
  [dt] -> Calculate Alpha1/1, Add1/1
  Compare To Zero4/1 -> Product2/1
  cutoff_freq/1 -> [cutoff_freq]
  Compare To Zero2/1 -> Logical Operator1/1
  [cutoff_freq] -> Compare To Zero3/1
  Calculate Alpha1/1 -> Switch1/3
  Logical Operator1/1 -> Switch1/2
  Constant5/1 -> Product2/2

== system arducopter/Rate Controller/PID Roll Rate/RAT_FLTE ==
  note: Digital Filter:
      | $y_n = (1 - \alpha)y_{n-1} + x \cdot \alpha$
  note: See AC_PID.cpp, update_all()
  note: See AP_Math.cpp, calc_lowpass_alpha_dt()
  note: Alpha Calculation:
      | $\alpha = \frac{\mathrm{d}t}{\mathrm{d}t + 2 \pi f_{\mathrm{Cutoff}}$
  u : Inport
  cutoff_freq : Inport  Port=2
  ATC input time constant1 : Constant  Value=simIn.param.dt
  Add1 : Sum
  Calculate Alpha1 : Product  Inputs=*/
  Compare To Zero2 : simulink/Logic and Bit Operations/Compare To Zero  relop=<=  OutDataTypeStr=boolean
  Compare To Zero3 : simulink/Logic and Bit Operations/Compare To Zero  relop=<=  OutDataTypeStr=boolean
  Compare To Zero4 : simulink/Logic and Bit Operations/Compare To Zero  relop=~=  OutDataTypeStr=boolean
  Constant1 : Constant  OutDataTypeStr=single
  Constant2 : Constant  OutDataTypeStr=single
  Constant5 : Constant  OutDataTypeStr=single
  Data Type Conversion1 : DataTypeConversion  OutDataTypeStr=single  SaturateOnIntegerOverflow=off  RndMeth=Floor
  Divide1 : Product  Inputs=*/
  Gain1 : Gain  Gain=2*pi
  IC : InitialCondition  Value=simIn.init.PIDR.ErrFilt
  Logical Operator1 : Logic  Operator=OR  AllPortsSameDT=off  OutDataTypeStr=boolean
  Product : Product
  Product1 : Product
  Product2 : Product
  Subtract1 : Sum  Inputs=+-
  Sum : Sum  Inputs=++|  OutDataTypeStr=single
  Switch1 : Switch  Criteria=u2 > Threshold  SaturateOnIntegerOverflow=off  InputSameDT=off
  Unit Delay : UnitDelay  SampleTime=-1  HasFrameUpgradeWarning=on
  y : Outport
  wires:
  Product1/1 -> Sum/2
  Unit Delay/1 -> Product1/2
  Subtract1/1 -> Product1/1
  [alpha] -> Subtract1/2
  Constant2/1 -> Subtract1/1
  [alpha] -> Product/1
  u/1 -> Product/2
  Product/1 -> Sum/1
  Sum/1 -> IC/1
  IC/1 -> Unit Delay/1, y/1
  [dt] -> Compare To Zero2/1
  Constant1/1 -> Divide1/1
  Divide1/1 -> Add1/2
  Product2/1 -> Switch1/1
  Add1/1 -> Calculate Alpha1/2
  Gain1/1 -> Divide1/2
  Compare To Zero3/1 -> Logical Operator1/2
  [dt] -> Compare To Zero4/1
  Data Type Conversion1/1 -> [dt]
  ATC input time constant1/1 -> Data Type Conversion1/1
  [cutoff_freq] -> Gain1/1
  Switch1/1 -> [alpha]
  [dt] -> Calculate Alpha1/1, Add1/1
  Compare To Zero4/1 -> Product2/1
  cutoff_freq/1 -> [cutoff_freq]
  Compare To Zero2/1 -> Logical Operator1/1
  [cutoff_freq] -> Compare To Zero3/1
  Calculate Alpha1/1 -> Switch1/3
  Logical Operator1/1 -> Switch1/2
  Constant5/1 -> Product2/2

== system arducopter/Rate Controller/PID Roll Rate/RAT_FLTT ==
  note: See AC_PID.cpp, update_all()
  note: Digital Filter:
      | $y_n = (1 - \alpha)y_{n-1} + x \cdot \alpha$
  note: Alpha Calculation:
      | $\alpha = \frac{\mathrm{d}t}{\mathrm{d}t + 2 \pi f_{\mathrm{Cutoff}}$
  note: See AP_Math.cpp, calc_lowpass_alpha_dt()
  u : Inport
  cutoff_freq : Inport  Port=2
  ATC input time constant1 : Constant  Value=simIn.param.dt
  Add1 : Sum
  Calculate Alpha1 : Product  Inputs=*/
  Compare To Zero2 : simulink/Logic and Bit Operations/Compare To Zero  relop=<=  OutDataTypeStr=boolean
  Compare To Zero3 : simulink/Logic and Bit Operations/Compare To Zero  relop=<=  OutDataTypeStr=boolean
  Compare To Zero4 : simulink/Logic and Bit Operations/Compare To Zero  relop=~=  OutDataTypeStr=boolean
  Constant1 : Constant  OutDataTypeStr=single
  Constant2 : Constant  OutDataTypeStr=single
  Constant5 : Constant  OutDataTypeStr=single
  Data Type Conversion1 : DataTypeConversion  OutDataTypeStr=single  SaturateOnIntegerOverflow=off  RndMeth=Floor
  Divide1 : Product  Inputs=*/
  Gain1 : Gain  Gain=2*pi
  IC : InitialCondition  Value=simIn.init.PIDR.TarFilt
  Logical Operator1 : Logic  Operator=OR  AllPortsSameDT=off  OutDataTypeStr=boolean
  Product : Product
  Product1 : Product
  Product2 : Product
  Subtract1 : Sum  Inputs=+-
  Sum : Sum  Inputs=++|
  Switch1 : Switch  Criteria=u2 > Threshold  SaturateOnIntegerOverflow=off  InputSameDT=off
  Unit Delay : UnitDelay  SampleTime=-1  HasFrameUpgradeWarning=on
  y : Outport
  wires:
  Product/1 -> Sum/1
  u/1 -> Product/2
  [alpha] -> Product/1
  Constant2/1 -> Subtract1/1
  [alpha] -> Subtract1/2
  Subtract1/1 -> Product1/1
  Product1/1 -> Sum/2
  Sum/1 -> IC/1
  Unit Delay/1 -> Product1/2
  IC/1 -> y/1, Unit Delay/1
  Add1/1 -> Calculate Alpha1/2
  Constant1/1 -> Divide1/1
  Compare To Zero2/1 -> Logical Operator1/1
  Logical Operator1/1 -> Switch1/2
  cutoff_freq/1 -> [cutoff_freq]
  Switch1/1 -> [alpha]
  [dt] -> Calculate Alpha1/1, Add1/1
  [cutoff_freq] -> Compare To Zero3/1
  Compare To Zero3/1 -> Logical Operator1/2
  Data Type Conversion1/1 -> [dt]
  [cutoff_freq] -> Gain1/1
  [dt] -> Compare To Zero2/1
  Divide1/1 -> Add1/2
  Gain1/1 -> Divide1/2
  ATC input time constant1/1 -> Data Type Conversion1/1
  Calculate Alpha1/1 -> Switch1/3
  [dt] -> Compare To Zero4/1
  Product2/1 -> Switch1/1
  Constant5/1 -> Product2/2
  Compare To Zero4/1 -> Product2/1

== system arducopter/Rate Controller/PID Roll Rate/Slew Limiter ==
  note: Data Store Memory Elements: Global variables of subsystem
  note: Slew Limiter
      |
      | Calculates the slew limit modifiert Dmod for the P and D part of the controller. The calculation of Dmod is taken from SlewLimiter::modifier() in SlewLimiter.cpp.
  note: Alpha Calculation:
      | $\alpha = \frac{\mathrm{d}t}{\mathrm{d}t + 2 \pi f_{\mathrm{Cutoff}}$
  note: See AP_Math.cpp, calc_lowpass_alpha_dt()
  p_out : Inport
  sr_max : Inport  Port=2
  sr_tau : Inport  Port=3
  sr_flt_f : Inport  Port=4
  clock : Inport  Port=5
  d_out : Inport  Port=6
  ATC input time constant : Constant  Value=simIn.param.dt
  Add1 : Sum
  Calculate Alpha : Product  Inputs=*/
  Calculate Dmod : MATLAB Function  TreatAsAtomicUnit=on  SystemSampleTime=0.0025
  Compare To Zero2 : simulink/Logic and Bit Operations/Compare To Zero  relop=<=  OutDataTypeStr=boolean
  Compare To Zero3 : simulink/Logic and Bit Operations/Compare To Zero  relop=<=  OutDataTypeStr=boolean
  Compare To Zero4 : simulink/Logic and Bit Operations/Compare To Zero  relop=~=  OutDataTypeStr=boolean
  Constant1 : Constant  OutDataTypeStr=single
  Constant5 : Constant  OutDataTypeStr=single
  Data Store Memory : DataStoreMemory  DataStoreName=pos_event_stored  ReadBeforeWriteMsg=warning  WriteAfterWriteMsg=warning  WriteAfterReadMsg=warning  InitialValue=false  ShowAdditionalParam=off  OutDataTypeStr=boolean
  Data Store Memory1 : DataStoreMemory  DataStoreName=neg_event_stored  ReadBeforeWriteMsg=warning  WriteAfterWriteMsg=warning  WriteAfterReadMsg=warning  InitialValue=false  ShowAdditionalParam=off  OutDataTypeStr=boolean
  Data Store Memory10 : DataStoreMemory  DataStoreName=modifier_slew_rate  ReadBeforeWriteMsg=warning  WriteAfterWriteMsg=warning  WriteAfterReadMsg=warning  InitialValue=simIn.init.PIDR.SROut  ShowAdditionalParam=off  OutDataTypeStr=single
  Data Store Memory11 : DataStoreMemory  DataStoreName=output_slew_rate  ReadBeforeWriteMsg=warning  WriteAfterWriteMsg=warning  WriteAfterReadMsg=warning  InitialValue=simIn.init.PIDR.SROut  ShowAdditionalParam=off  OutDataTypeStr=single
  Data Store Memory2 : DataStoreMemory  DataStoreName=pos_event_idx  ReadBeforeWriteMsg=warning  WriteAfterWriteMsg=warning  WriteAfterReadMsg=warning  InitialValue=1  ShowAdditionalParam=off  OutDataTypeStr=int8
  Data Store Memory3 : DataStoreMemory  DataStoreName=neg_event_idx  ReadBeforeWriteMsg=warning  WriteAfterWriteMsg=warning  WriteAfterReadMsg=warning  InitialValue=1  ShowAdditionalParam=off  OutDataTypeStr=int8
  Data Store Memory4 : DataStoreMemory  DataStoreName=pos_event_ms  ReadBeforeWriteMsg=warning  WriteAfterWriteMsg=warning  WriteAfterReadMsg=warning  InitialValue=[0 0]  ShowAdditionalParam=off  OutDataTypeStr=uint32  Dimensions=2
  Data Store Memory5 : DataStoreMemory  DataStoreName=neg_event_ms  ReadBeforeWriteMsg=warning  WriteAfterWriteMsg=warning  WriteAfterReadMsg=warning  InitialValue=[0 0]  ShowAdditionalParam=off  OutDataTypeStr=uint32  Dimensions=2
  Data Store Memory6 : DataStoreMemory  DataStoreName=max_pos_slew_rate  ReadBeforeWriteMsg=warning  WriteAfterWriteMsg=warning  WriteAfterReadMsg=warning  ShowAdditionalParam=off  OutDataTypeStr=single
  Data Store Memory7 : DataStoreMemory  DataStoreName=max_pos_slew_event_ms  ReadBeforeWriteMsg=warning  WriteAfterWriteMsg=warning  WriteAfterReadMsg=warning  ShowAdditionalParam=off  OutDataTypeStr=uint32
  Data Store Memory8 : DataStoreMemory  DataStoreName=max_neg_slew_rate  ReadBeforeWriteMsg=warning  WriteAfterWriteMsg=warning  WriteAfterReadMsg=warning  ShowAdditionalParam=off  OutDataTypeStr=single
  Data Store Memory9 : DataStoreMemory  DataStoreName=max_neg_slew_event_ms  ReadBeforeWriteMsg=warning  WriteAfterWriteMsg=warning  WriteAfterReadMsg=warning  ShowAdditionalParam=off  OutDataTypeStr=uint32
  Data Store Read : DataStoreRead  DataStoreName=modifier_slew_rate  DataStoreElements=modifier_slew_rate  IndexOptions=Index vector (dialog)  Indices=1  OutputSizes=1
  Data Store Read1 : DataStoreRead  DataStoreName=output_slew_rate  DataStoreElements=output_slew_rate  IndexOptions=Index vector (dialog)  Indices=1  OutputSizes=1
  Data Type Conversion2 : DataTypeConversion  OutDataTypeStr=single  SaturateOnIntegerOverflow=off  RndMeth=Floor
  Divide1 : Product  Inputs=*/
  Gain1 : Gain  Gain=2*pi
  IC : InitialCondition  Value=2*simIn.init.PIDR.SROut
  Logical Operator1 : Logic  Operator=OR  AllPortsSameDT=off  OutDataTypeStr=boolean
  Lowpass Filter : MATLAB Function  TreatAsAtomicUnit=on
  Product2 : Product
  Subsystem : Subsystem
  Switch1 : Switch  Criteria=u2 > Threshold  SaturateOnIntegerOverflow=off  InputSameDT=off
  Terminator : Terminator
  Terminator1 : Terminator
  Unit Delay1 : UnitDelay  SampleTime=-1  HasFrameUpgradeWarning=on
  Dmod : Outport
  wires:
  Lowpass Filter/1(out) -> IC/1  "rollRateSrFilt"
  Unit Delay1/1 -> Lowpass Filter/3(out_last)
  Calculate Dmod/1(Dmod) -> Dmod/1  "rollRateDmod"
  sr_max/1 -> Calculate Dmod/2(sr_max)
  sr_tau/1 -> Calculate Dmod/3(sr_tau)
  Data Store Read/1 -> Terminator/1  "rollRateSrModifier"
  Data Store Read1/1 -> Terminator1/1  "rollRateSrOut"
  p_out/1 -> Subsystem/1(p_out)
  d_out/1 -> Subsystem/2(d_out)
  Subsystem/1(sr_raw) -> Lowpass Filter/1(in)  "rollRateSrRaw"
  IC/1 -> Calculate Dmod/1(slew_rate), Unit Delay1/1
  clock/1 -> Calculate Dmod/5(time)
  [cutoff_freq] -> Gain1/1
  [dt] -> Calculate Alpha/1, Add1/1
  Calculate Alpha/1 -> Switch1/3
  Gain1/1 -> Divide1/2
  Data Type Conversion2/1 -> [dt]
  ATC input time constant/1 -> Data Type Conversion2/1
  [cutoff_freq] -> Compare To Zero3/1
  Compare To Zero3/1 -> Logical Operator1/2
  Constant1/1 -> Divide1/1
  [dt] -> Compare To Zero2/1
  Logical Operator1/1 -> Switch1/2
  Compare To Zero2/1 -> Logical Operator1/1
  Add1/1 -> Calculate Alpha/2
  Divide1/1 -> Add1/2
  Product2/1 -> Switch1/1
  [dt] -> Compare To Zero4/1
  Switch1/1 -> Lowpass Filter/2(alpha)
  Compare To Zero4/1 -> Product2/1
  Constant5/1 -> Product2/2
  sr_flt_f/1 -> [cutoff_freq]
  [dt] -> Calculate Dmod/4(dt)

== system arducopter/Rate Controller/PID Yaw Rate/Calc Derivative ==
  e : Inport
  ATC input time constant : Constant  Value=simIn.param.dt
  Data Type Conversion : DataTypeConversion  OutDataTypeStr=single  SaturateOnIntegerOverflow=off  RndMeth=Floor
  Divide : Product  Inputs=*/
  Sum : Sum  Inputs=|+-
  Unit Delay : UnitDelay  SampleTime=-1  HasFrameUpgradeWarning=on
  derivative : Outport
  wires:
  e/1 -> Sum/1, Unit Delay/1
  Unit Delay/1 -> Sum/2
  Sum/1 -> Divide/1
  ATC input time constant/1 -> Data Type Conversion/1
  Divide/1 -> derivative/1
  Data Type Conversion/1 -> Divide/2

== system arducopter/Rate Controller/PID Yaw Rate/I ==
  note: Integrator, see AC_PID::update_i()
  e : Inport
  limit_flg : Inport  Port=2
  ki : Inport  Port=3
  i_max : Inport  Port=4
  Constant1 : Constant  Value=simIn.param.dt
  Data Type Conversion : DataTypeConversion  OutDataTypeStr=single  SaturateOnIntegerOverflow=off  RndMeth=Floor
  IC1 : InitialCondition  Value=simIn.init.PIDY.I
  Integrator : MATLAB Function  TreatAsAtomicUnit=on
  Unit Delay1 : UnitDelay  SampleTime=-1  HasFrameUpgradeWarning=on
  integrator : Outport
  wires:
  [integrator_out] -> integrator/1
  Constant1/1 -> Data Type Conversion/1
  limit_flg/1 -> Integrator/3(limit_flg)
  [integrator_out] -> Unit Delay1/1
  IC1/1 -> [integrator_out]
  Unit Delay1/1 -> Integrator/2(integrator)
  ki/1 -> Integrator/4(ki)
  i_max/1 -> Integrator/5(i_max)
  e/1 -> Integrator/1(error)
  Integrator/1(integrator_out) -> IC1/1
  Data Type Conversion/1 -> Integrator/6(dt)

== system arducopter/Rate Controller/PID Yaw Rate/RAT_FLTD ==
  note: Digital Filter:
      | $y_n = (1 - \alpha)y_{n-1} + x \cdot \alpha$
  note: See AC_PID.cpp, update_all()
  note: See AP_Math.cpp, calc_lowpass_alpha_dt()
  note: Alpha Calculation:
      | $\alpha = \frac{\mathrm{d}t}{\mathrm{d}t + 2 \pi f_{\mathrm{Cutoff}}$
  u : Inport
  cutoff_freq : Inport  Port=2
  ATC input time constant1 : Constant  Value=simIn.param.dt
  Add1 : Sum
  Calculate Alpha1 : Product  Inputs=*/
  Compare To Zero2 : simulink/Logic and Bit Operations/Compare To Zero  relop=<=  OutDataTypeStr=boolean
  Compare To Zero3 : simulink/Logic and Bit Operations/Compare To Zero  relop=<=  OutDataTypeStr=boolean
  Compare To Zero4 : simulink/Logic and Bit Operations/Compare To Zero  relop=~=  OutDataTypeStr=boolean
  Constant1 : Constant  OutDataTypeStr=single
  Constant2 : Constant  OutDataTypeStr=single
  Constant5 : Constant  OutDataTypeStr=single
  Data Type Conversion1 : DataTypeConversion  OutDataTypeStr=single  SaturateOnIntegerOverflow=off  RndMeth=Floor
  Divide1 : Product  Inputs=*/
  Gain1 : Gain  Gain=2*pi
  IC : InitialCondition  Value=simIn.init.PIDY.DerFilt
  Logical Operator1 : Logic  Operator=OR  AllPortsSameDT=off  OutDataTypeStr=boolean
  Product : Product
  Product1 : Product
  Product2 : Product
  Subtract1 : Sum  Inputs=+-
  Sum : Sum  Inputs=++|  AccumDataTypeStr=single
  Switch1 : Switch  Criteria=u2 > Threshold  SaturateOnIntegerOverflow=off  InputSameDT=off
  Unit Delay : UnitDelay  SampleTime=-1  HasFrameUpgradeWarning=on
  y : Outport
  wires:
  Product1/1 -> Sum/2
  Unit Delay/1 -> Product1/2
  Subtract1/1 -> Product1/1
  [alpha] -> Subtract1/2
  Constant2/1 -> Subtract1/1
  [alpha] -> Product/1
  u/1 -> Product/2
  Product/1 -> Sum/1
  Sum/1 -> IC/1
  IC/1 -> Unit Delay/1, y/1
  [dt] -> Compare To Zero2/1
  Constant1/1 -> Divide1/1
  Divide1/1 -> Add1/2
  Product2/1 -> Switch1/1
  Add1/1 -> Calculate Alpha1/2
  Gain1/1 -> Divide1/2
  Compare To Zero3/1 -> Logical Operator1/2
  [dt] -> Compare To Zero4/1
  Data Type Conversion1/1 -> [dt]
  ATC input time constant1/1 -> Data Type Conversion1/1
  [cutoff_freq] -> Gain1/1
  Switch1/1 -> [alpha]
  [dt] -> Calculate Alpha1/1, Add1/1
  Compare To Zero4/1 -> Product2/1
  cutoff_freq/1 -> [cutoff_freq]
  Compare To Zero2/1 -> Logical Operator1/1
  [cutoff_freq] -> Compare To Zero3/1
  Calculate Alpha1/1 -> Switch1/3
  Logical Operator1/1 -> Switch1/2
  Constant5/1 -> Product2/2

== system arducopter/Rate Controller/PID Yaw Rate/RAT_FLTE ==
  note: Digital Filter:
      | $y_n = (1 - \alpha)y_{n-1} + x \cdot \alpha$
  note: See AC_PID.cpp, update_all()
  note: See AP_Math.cpp, calc_lowpass_alpha_dt()
  note: Alpha Calculation:
      | $\alpha = \frac{\mathrm{d}t}{\mathrm{d}t + 2 \pi f_{\mathrm{Cutoff}}$
  u : Inport
  cutoff_freq : Inport  Port=2
  ATC input time constant1 : Constant  Value=simIn.param.dt
  Add1 : Sum
  Calculate Alpha1 : Product  Inputs=*/
  Compare To Zero2 : simulink/Logic and Bit Operations/Compare To Zero  relop=<=  OutDataTypeStr=boolean
  Compare To Zero3 : simulink/Logic and Bit Operations/Compare To Zero  relop=<=  OutDataTypeStr=boolean
  Compare To Zero4 : simulink/Logic and Bit Operations/Compare To Zero  relop=~=  OutDataTypeStr=boolean
  Constant1 : Constant  OutDataTypeStr=single
  Constant2 : Constant  OutDataTypeStr=single
  Constant5 : Constant  OutDataTypeStr=single
  Data Type Conversion1 : DataTypeConversion  OutDataTypeStr=single  SaturateOnIntegerOverflow=off  RndMeth=Floor
  Divide1 : Product  Inputs=*/
  Gain1 : Gain  Gain=2*pi
  IC : InitialCondition  Value=simIn.init.PIDY.ErrFilt
  Logical Operator1 : Logic  Operator=OR  AllPortsSameDT=off  OutDataTypeStr=boolean
  Product : Product
  Product1 : Product
  Product2 : Product
  Subtract1 : Sum  Inputs=+-
  Sum : Sum  Inputs=++|  OutDataTypeStr=single
  Switch1 : Switch  Criteria=u2 > Threshold  SaturateOnIntegerOverflow=off  InputSameDT=off
  Unit Delay : UnitDelay  SampleTime=-1  HasFrameUpgradeWarning=on
  y : Outport
  wires:
  Product1/1 -> Sum/2
  Unit Delay/1 -> Product1/2
  Subtract1/1 -> Product1/1
  [alpha] -> Subtract1/2
  Constant2/1 -> Subtract1/1
  [alpha] -> Product/1
  u/1 -> Product/2
  Product/1 -> Sum/1
  Sum/1 -> IC/1
  IC/1 -> Unit Delay/1, y/1
  [dt] -> Compare To Zero2/1
  Constant1/1 -> Divide1/1
  Divide1/1 -> Add1/2
  Product2/1 -> Switch1/1
  Add1/1 -> Calculate Alpha1/2
  Gain1/1 -> Divide1/2
  Compare To Zero3/1 -> Logical Operator1/2
  [dt] -> Compare To Zero4/1
  Data Type Conversion1/1 -> [dt]
  ATC input time constant1/1 -> Data Type Conversion1/1
  [cutoff_freq] -> Gain1/1
  Switch1/1 -> [alpha]
  [dt] -> Calculate Alpha1/1, Add1/1
  Compare To Zero4/1 -> Product2/1
  cutoff_freq/1 -> [cutoff_freq]
  Compare To Zero2/1 -> Logical Operator1/1
  [cutoff_freq] -> Compare To Zero3/1
  Calculate Alpha1/1 -> Switch1/3
  Logical Operator1/1 -> Switch1/2
  Constant5/1 -> Product2/2

== system arducopter/Rate Controller/PID Yaw Rate/RAT_FLTT ==
  note: See AC_PID.cpp, update_all()
  note: Digital Filter:
      | $y_n = (1 - \alpha)y_{n-1} + x \cdot \alpha$
  note: Alpha Calculation:
      | $\alpha = \frac{\mathrm{d}t}{\mathrm{d}t + 2 \pi f_{\mathrm{Cutoff}}$
  note: See AP_Math.cpp, calc_lowpass_alpha_dt()
  u : Inport
  cutoff_freq : Inport  Port=2
  ATC input time constant1 : Constant  Value=simIn.param.dt
  Add1 : Sum
  Calculate Alpha1 : Product  Inputs=*/
  Compare To Zero2 : simulink/Logic and Bit Operations/Compare To Zero  relop=<=  OutDataTypeStr=boolean
  Compare To Zero3 : simulink/Logic and Bit Operations/Compare To Zero  relop=<=  OutDataTypeStr=boolean
  Compare To Zero4 : simulink/Logic and Bit Operations/Compare To Zero  relop=~=  OutDataTypeStr=boolean
  Constant1 : Constant  OutDataTypeStr=single
  Constant2 : Constant  OutDataTypeStr=single
  Constant5 : Constant  OutDataTypeStr=single
  Data Type Conversion1 : DataTypeConversion  OutDataTypeStr=single  SaturateOnIntegerOverflow=off  RndMeth=Floor
  Divide1 : Product  Inputs=*/
  Gain1 : Gain  Gain=2*pi
  IC : InitialCondition  Value=simIn.init.PIDY.TarFilt
  Logical Operator1 : Logic  Operator=OR  AllPortsSameDT=off  OutDataTypeStr=boolean
  Product : Product
  Product1 : Product
  Product2 : Product
  Subtract1 : Sum  Inputs=+-
  Sum : Sum  Inputs=++|
  Switch1 : Switch  Criteria=u2 > Threshold  SaturateOnIntegerOverflow=off  InputSameDT=off
  Unit Delay : UnitDelay  SampleTime=-1  HasFrameUpgradeWarning=on
  y : Outport
  wires:
  Product/1 -> Sum/1
  u/1 -> Product/2
  [alpha] -> Product/1
  Constant2/1 -> Subtract1/1
  [alpha] -> Subtract1/2
  Subtract1/1 -> Product1/1
  Product1/1 -> Sum/2
  Sum/1 -> IC/1
  Unit Delay/1 -> Product1/2
  IC/1 -> y/1, Unit Delay/1
  Add1/1 -> Calculate Alpha1/2
  Constant1/1 -> Divide1/1
  Compare To Zero2/1 -> Logical Operator1/1
  Logical Operator1/1 -> Switch1/2
  cutoff_freq/1 -> [cutoff_freq]
  Switch1/1 -> [alpha]
  [dt] -> Calculate Alpha1/1, Add1/1
  [cutoff_freq] -> Compare To Zero3/1
  Compare To Zero3/1 -> Logical Operator1/2
  Data Type Conversion1/1 -> [dt]
  [cutoff_freq] -> Gain1/1
  [dt] -> Compare To Zero2/1
  Divide1/1 -> Add1/2
  Gain1/1 -> Divide1/2
  ATC input time constant1/1 -> Data Type Conversion1/1
  Calculate Alpha1/1 -> Switch1/3
  [dt] -> Compare To Zero4/1
  Product2/1 -> Switch1/1
  Constant5/1 -> Product2/2
  Compare To Zero4/1 -> Product2/1
